simulink model "ADCS_v1"  (R2026a)
settings: Solver=VariableStepAuto  StopTime=t0  FixedStep=0.1  MaxStep=0.1
model workspace (MAT data in the model file):
  i = 8
  omega_thr = 1
  simIn : Simulink.SimulationInput (value not decoded)
  t = [0 0.1 0.2 0.3 0.4 0.5 0.6 0.7 0.8 0.9 1 1.1 ... (101 elements, 101x1)]
  u : object (value not decoded)
  y_out = [0 0 0 0 0 0 0 0]
values from neighbouring files (symbols this model uses):
  B = [1 0 0]    [parameters.m]
  h_max = 1.47    [parameters.m]
  I_RW = 1    [parameters.m]
  k_desat = 1    [parameters.m]
  kd_detumble = 1    [parameters.m]
  kd_hold = 1    [parameters.m]
  kd_point = 20    [parameters.m]
  kd_slew_fast = 1    [parameters.m]
  kd_slew_slow = 1    [parameters.m]
  kd_spin = 0    [parameters.m]
  kp_hold = 1    [parameters.m]
  kp_point = 2    [parameters.m]
  kp_slew_fast = 1    [parameters.m]
  kp_slew_slow = 1    [parameters.m]
  kp_spin = 1    [parameters.m]
  omega_0 = [0 0 0.0011]    [parameters.m]
  omega_ref = [0 0 0]    [parameters.m]
  omega_zero = 0.001    [parameters.m]
  P = satellite_params()    [individual_test_with_dynamics.m]    (also in parameters.m; test.m = thrusters(:, 1:3))
  q0 = [sqrt(0.5) -sqrt(0.5) 0 0]    [parameters.m]
  q_ref = [ cos(theta_ref/2) ... (first row only)    [parameters.m]
libraries: matrix_library x13, simulink x6, aerolibutil x4, sim3dlib x2
(part 2 of 2)

== system ADCS_v1/Subsystem2/Controller/Subsystem ==
  q_ref : Inport
  q : Inport  Port=2
  omega_ref : Inport  Port=3
  omega : Inport  Port=4
  Quaternion Inverse : aerolibutil/Quaternion Inverse
  Quaternion Multiplication : aerolibutil/Quaternion Multiplication
  Sum : Sum  Inputs=|+-
  Terminator : Terminator
  split q_error : Demux  Outputs=[1 3]
  q_err : Outport
  omega_err : Outport  Port=2
  wires:
  omega_ref/1 -> Sum/2
  omega/1 -> Sum/1
  Quaternion Inverse/1 -> Quaternion Multiplication/1
  q_ref/1 -> Quaternion Multiplication/2
  split q_error/1 -> Terminator/1
  split q_error/2 -> q_err/1
  Quaternion Multiplication/1 -> split q_error/1
  Sum/1 -> omega_err/1
  q/1 -> Quaternion Inverse/1

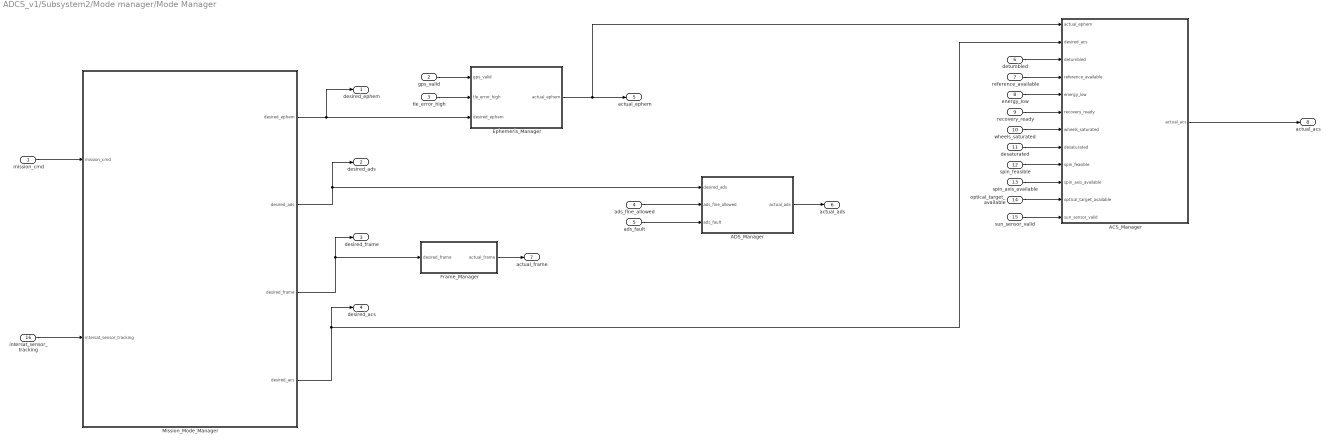
== system ADCS_v1/Subsystem2/Mode manager/Mode Manager ==
  mission_cmd : Inport  OutDataTypeStr=uint8  PortDimensions=1
  gps_valid : Inport  Port=2  OutDataTypeStr=boolean  PortDimensions=1
  tle_error_high : Inport  Port=3  OutDataTypeStr=boolean  PortDimensions=1
  ads_fine_allowed : Inport  Port=4  OutDataTypeStr=boolean  PortDimensions=1
  ads_fault : Inport  Port=5  OutDataTypeStr=boolean  PortDimensions=1
  detumbled : Inport  Port=6  OutDataTypeStr=boolean  PortDimensions=1
  reference_available : Inport  Port=7  OutDataTypeStr=boolean  PortDimensions=1
  energy_low : Inport  Port=8  OutDataTypeStr=boolean  PortDimensions=1
  recovery_ready : Inport  Port=9  OutDataTypeStr=boolean  PortDimensions=1
  wheels_saturated : Inport  Port=10  OutDataTypeStr=boolean  PortDimensions=1
  desaturated : Inport  Port=11  OutDataTypeStr=boolean  PortDimensions=1
  spin_feasible : Inport  Port=12  OutDataTypeStr=boolean  PortDimensions=1
  spin_axis_available : Inport  Port=13  OutDataTypeStr=boolean  PortDimensions=1
  optical_target_available : Inport  Port=14  OutDataTypeStr=boolean  PortDimensions=1
  sun_sensor_valid : Inport  Port=15  OutDataTypeStr=boolean  PortDimensions=1
  intersat_sensor_tracking : Inport  Port=16  OutDataTypeStr=boolean  PortDimensions=1
  ACS_Manager : Stateflow chart  TreatAsAtomicUnit=on
      settings: PortSchema="{\"entries\":[{\"content\":{\"sides\":[{\"content\":{\"connectorIds\":[\"In2\",\"In1\",\"In3\",\"In4\",\"In5\",\"In6\",\"In7\",\"In8\",\"In9\",\"In10\",\"In11\",\"In12\"]},\"type\":\"ConnectorPlacement.EquallySpacedRectSide\",\"uuid\":\"c64f5ed7-7a07-4761-a251-d625087249f8\"},{\"content\":{\"connectorIds\":[\"Out1\"],\"side\":\"RIGHT\"},\"type\":\"ConnectorPlacement.EquallySpacedRectSide\",\"uuid\":\"ff17dfa7-5a32-4799-bec0-131df3b46d45\"},{\"content\":{\"side\":\"TOP\"},\"type\":\"ConnectorPlacement.EquallySpacedRectSide\",\"uuid\":\"acaf274e-12ec-4fab-ab7e-ad580afcef6e\"}]},\"type\":\"ConnectorPlacement.EquallySpacedConnector\",\"uuid\":\"7d19de63-b993-417e-b6e9-9dc888da130b\"}],\"packageUris\":[\"http://schema.mathworks.com/mf0/Connector/R2020b\"],\"version\":\"1.0\"}"
  ADS_Manager : Stateflow chart  TreatAsAtomicUnit=on
  Ephemeris_Manager : Stateflow chart  TreatAsAtomicUnit=on
      settings: PortSchema="{\"entries\":[{\"content\":{\"sides\":[{\"content\":{\"connectorIds\":[\"In2\",\"In3\",\"In1\"]},\"type\":\"ConnectorPlacement.EquallySpacedRectSide\",\"uuid\":\"cbbccf67-8c60-498d-a98a-76db8747fb3a\"},{\"content\":{\"connectorIds\":[\"Out1\"],\"side\":\"RIGHT\"},\"type\":\"ConnectorPlacement.EquallySpacedRectSide\",\"uuid\":\"743b35d2-d398-4833-9c20-93b5e77612f2\"},{\"content\":{\"side\":\"TOP\"},\"type\":\"ConnectorPlacement.EquallySpacedRectSide\",\"uuid\":\"56075cc1-c683-438a-85bf-78d94186ffa6\"}]},\"type\":\"ConnectorPlacement.EquallySpacedConnector\",\"uuid\":\"bae867d4-09fc-4097-a23b-eff5fb3633ac\"}],\"packageUris\":[\"http://schema.mathworks.com/mf0/Connector/R2020b\"],\"version\":\"1.0\"}"
  Frame_Manager : Stateflow chart  TreatAsAtomicUnit=on
  Mission_Mode_Manager : Stateflow chart  TreatAsAtomicUnit=on
  desired_ephem : Outport
  desired_ads : Outport  Port=2
  desired_frame : Outport  Port=3
  desired_acs : Outport  Port=4
  actual_ephem : Outport  Port=5
  actual_ads : Outport  Port=6
  actual_frame : Outport  Port=7
  actual_acs : Outport  Port=8
  wires:
  spin_feasible/1 -> ACS_Manager/9(spin_feasible)
  desaturated/1 -> ACS_Manager/8(desaturated)
  spin_axis_available/1 -> ACS_Manager/10(spin_axis_available)
  mission_cmd/1 -> Mission_Mode_Manager/1(mission_cmd)
  recovery_ready/1 -> ACS_Manager/6(recovery_ready)
  ads_fault/1 -> ADS_Manager/3(ads_fault)
  intersat_sensor_tracking/1 -> Mission_Mode_Manager/2(intersat_sensor_tracking)
  gps_valid/1 -> Ephemeris_Manager/2(gps_valid)
  Ephemeris_Manager/1(actual_ephem) -> ACS_Manager/2(actual_ephem), actual_ephem/1
  ads_fine_allowed/1 -> ADS_Manager/2(ads_fine_allowed)
  ADS_Manager/1(actual_ads) -> actual_ads/1
  Mission_Mode_Manager/3(desired_frame) -> Frame_Manager/1(desired_frame), desired_frame/1
  wheels_saturated/1 -> ACS_Manager/7(wheels_saturated)
  detumbled/1 -> ACS_Manager/3(detumbled)
  reference_available/1 -> ACS_Manager/4(reference_available)
  tle_error_high/1 -> Ephemeris_Manager/3(tle_error_high)
  Mission_Mode_Manager/2(desired_ads) -> ADS_Manager/1(desired_ads), desired_ads/1
  optical_target_available/1 -> ACS_Manager/11(optical_target_available)
  Frame_Manager/1(actual_frame) -> actual_frame/1
  Mission_Mode_Manager/1(desired_ephem) -> desired_ephem/1, Ephemeris_Manager/1(desired_ephem)
  energy_low/1 -> ACS_Manager/5(energy_low)
  Mission_Mode_Manager/4(desired_acs) -> desired_acs/1, ACS_Manager/1(desired_acs)
  ACS_Manager/1(actual_acs) -> actual_acs/1
  sun_sensor_valid/1 -> ACS_Manager/12(sun_sensor_valid)

== system ADCS_v1/Subsystem1/Controller/Control Algorithms/DESAT ==
  B : Inport
  RW_omega : Inport  Port=2
  desat : ActionPort
  Cross Product : matrix_library/Cross Product
  Divide : Product  Inputs=*/
  Dot Product : DotProduct  OutDataTypeStr=Inherit: Inherit via internal rule
  Gain : Gain  Gain=-k_desat
  tau_cmd : Outport
  wires:
  B/1 -> Dot Product/1, Dot Product/2, Cross Product/2
  Divide/1 -> Gain/1
  Gain/1 -> tau_cmd/1
  Cross Product/1 -> Divide/1
  RW_omega/1 -> Cross Product/1
  Dot Product/1 -> Divide/2

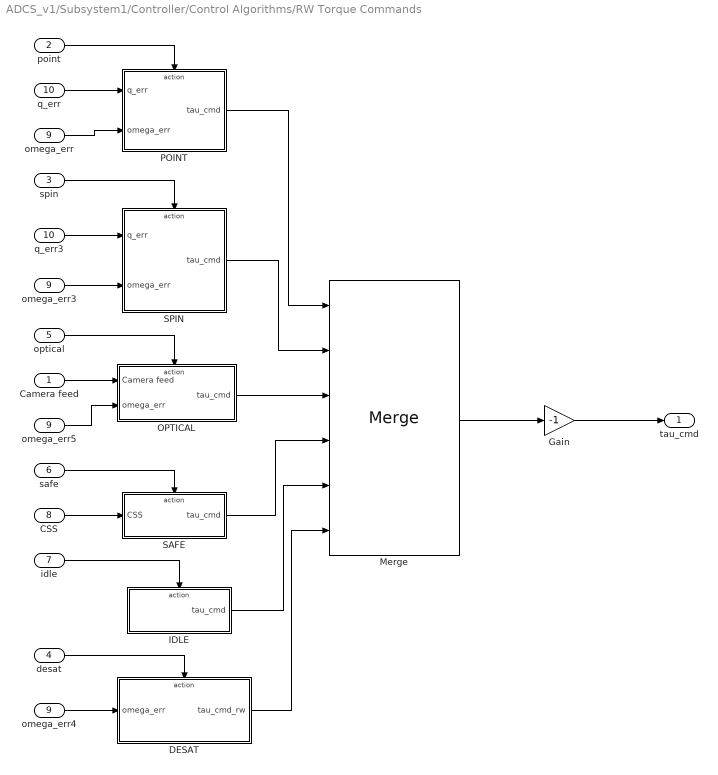
== system ADCS_v1/Subsystem1/Controller/Control Algorithms/RW Torque Commands ==
  Camera feed : Inport
  point : Inport  Port=2
  spin : Inport  Port=3
  desat : Inport  Port=4
  optical : Inport  Port=5
  safe : Inport  Port=6
  idle : Inport  Port=7
  CSS : Inport  Port=8
  omega_err : Inport  Port=9
  q_err : Inport  Port=10
  DESAT : Subsystem  TreatAsAtomicUnit=on
  Gain : Gain  Gain=-1
  IDLE : Subsystem  TreatAsAtomicUnit=on
  Merge : Merge  Inputs=6
  OPTICAL : Subsystem  TreatAsAtomicUnit=on
  POINT : Subsystem  TreatAsAtomicUnit=on
  SAFE : Subsystem  TreatAsAtomicUnit=on
  SPIN : Subsystem  TreatAsAtomicUnit=on
  omega_err3 : InportShadow  Port=9
  omega_err4 : InportShadow  Port=9
  omega_err5 : InportShadow  Port=9
  q_err3 : InportShadow  Port=10
  tau_cmd : Outport
  wires:
  idle/1 -> IDLE/Action
  spin/1 -> SPIN/Action
  Camera feed/1 -> OPTICAL/1(Camera feed)
  omega_err4/1 -> DESAT/1(omega_err)
  omega_err/1 -> POINT/2(omega_err)
  optical/1 -> OPTICAL/Action
  desat/1 -> DESAT/Action
  CSS/1 -> SAFE/1(CSS)
  point/1 -> POINT/Action
  omega_err3/1 -> SPIN/2(omega_err)
  safe/1 -> SAFE/Action
  q_err/1 -> POINT/1(q_err)
  q_err3/1 -> SPIN/1(q_err)
  omega_err5/1 -> OPTICAL/2(omega_err)
  POINT/1(tau_cmd) -> Merge/1
  SPIN/1(tau_cmd) -> Merge/2
  OPTICAL/1(tau_cmd) -> Merge/3
  SAFE/1(tau_cmd) -> Merge/4
  IDLE/1(tau_cmd) -> Merge/5
  DESAT/1(tau_cmd_rw) -> Merge/6
  Merge/1 -> Gain/1
  Gain/1 -> tau_cmd/1

== system ADCS_v1/Subsystem1/Controller/Control Algorithms/Thruster Torque commands ==
  detumble : Inport
  desat : Inport  Port=2
  default : Inport  Port=3
  omega : Inport  Port=4
  RW_omega : Inport  Port=5
  DEFAULT : Subsystem  TreatAsAtomicUnit=on
  DESAT : Subsystem  TreatAsAtomicUnit=on
  DETUMBLE : Subsystem  TreatAsAtomicUnit=on
  Merge1 : Merge  Inputs=3
  tau_cmd : Outport
  wires:
  omega/1 -> DETUMBLE/1(omega)
  DETUMBLE/1(tau_cmd) -> Merge1/1
  Merge1/1 -> tau_cmd/1
  detumble/1 -> DETUMBLE/Action
  default/1 -> DEFAULT/Action
  DEFAULT/1(tau_cmd) -> Merge1/3
  RW_omega/1 -> DESAT/1(RW_omega)
  desat/1 -> DESAT/Action
  DESAT/1(tau_cmd) -> Merge1/2

== system ADCS_v1/Subsystem1/Controller/Control Algorithms/default ==
  detumble : ActionPort
  Constant : Constant  Value=[0 0 0]
  tau_cmd : Outport
  wires:
  Constant/1 -> tau_cmd/1

== system ADCS_v1/Subsystem1/Subsystem/LVLH/norm ==
  In1 : Inport
  Sqrt : Sqrt
  Square : Math  Operator=square
  Sum of Elements : Sum  Inputs=+
  Out1 : Outport
  wires:
  In1/1 -> Square/1
  Square/1 -> Sum of Elements/1
  Sum of Elements/1 -> Sqrt/1
  Sqrt/1 -> Out1/1

== system ADCS_v1/Subsystem1/Subsystem/LVLH/norm1 ==
  In1 : Inport
  Sqrt : Sqrt
  Square : Math  Operator=square
  Sum of Elements : Sum  Inputs=+
  Out1 : Outport
  wires:
  Sqrt/1 -> Out1/1
  Sum of Elements/1 -> Sqrt/1
  Square/1 -> Sum of Elements/1
  In1/1 -> Square/1

== system ADCS_v1/Subsystem1/Subsystem/Sun_point/Pointing_r ==
  v_si : Inport
  r_si : Inport  Port=2
  v_sun_i : Inport  Port=3
  r_sun_i : Inport  Port=4
  Sum : Sum  Inputs=|-+
  Sum1 : Sum  Inputs=|-+
  v_point : Outport
  r_point : Outport  Port=2
  wires:
  Sum1/1 -> v_point/1
  v_si/1 -> Sum1/1
  Sum/1 -> r_point/1
  r_si/1 -> Sum/1
  v_sun_i/1 -> Sum1/2
  r_sun_i/1 -> Sum/2

== system ADCS_v1/Subsystem1/Subsystem/Sun_point/norm ==
  r_point : Inport
  Sqrt : Sqrt
  Square : Math  Operator=square
  Sum of Elements : Sum  Inputs=+
  Out1 : Outport
  wires:
  r_point/1 -> Square/1
  Square/1 -> Sum of Elements/1
  Sum of Elements/1 -> Sqrt/1
  Sqrt/1 -> Out1/1

== system ADCS_v1/Subsystem1/Subsystem/Sun_point/norm1 ==
  In1 : Inport
  Sqrt : Sqrt
  Square : Math  Operator=square
  Sum of Elements : Sum  Inputs=+
  Out1 : Outport
  wires:
  Sqrt/1 -> Out1/1
  Sum of Elements/1 -> Sqrt/1
  Square/1 -> Sum of Elements/1
  In1/1 -> Square/1

== system ADCS_v1/Subsystem1/Subsystem/Target_Pointing/Pointing_r ==
  v_si : Inport
  r_si : Inport  Port=2
  r_pi : Inport  Port=3
  Sum : Sum  Inputs=-+|
  Sum1 : Sum  Inputs=|-+
  omega_E : Constant  Value=[0 0 7.2921159e-5]
  v_p : matrix_library/Cross Product
  v_point : Outport
  r_point : Outport  Port=2
  wires:
  r_si/1 -> Sum/1
  r_pi/1 -> v_p/2, Sum/2
  Sum/1 -> r_point/1
  v_si/1 -> Sum1/1
  omega_E/1 -> v_p/1
  Sum1/1 -> v_point/1
  v_p/1 -> Sum1/2

== system ADCS_v1/Subsystem1/Subsystem/Target_Pointing/norm ==
  r_point : Inport
  Sqrt : Sqrt
  Square : Math  Operator=square
  Sum of Elements : Sum  Inputs=+
  Out1 : Outport
  wires:
  Sqrt/1 -> Out1/1
  Sum of Elements/1 -> Sqrt/1
  Square/1 -> Sum of Elements/1
  r_point/1 -> Square/1

== system ADCS_v1/Subsystem1/Subsystem/Target_Pointing/norm1 ==
  In1 : Inport
  Sqrt : Sqrt
  Square : Math  Operator=square
  Sum of Elements : Sum  Inputs=+
  Out1 : Outport
  wires:
  In1/1 -> Square/1
  Square/1 -> Sum of Elements/1
  Sum of Elements/1 -> Sqrt/1
  Sqrt/1 -> Out1/1

== system ADCS_v1/Subsystem1/Subsystem/VNB/Subsystem ==
  In1 : Inport
  Default : Subsystem  TreatAsAtomicUnit=on
  M_MAX_DRAG : Subsystem  TreatAsAtomicUnit=on
  M_MIN_DRAG : Subsystem  TreatAsAtomicUnit=on
  M_RAM : Subsystem  TreatAsAtomicUnit=on
  Merge : Merge  Inputs=4
  Switch Case : SwitchCase  CaseConditions={8,9,10}
  Out3 : Outport
  wires:
  Switch Case/1 -> M_MIN_DRAG/Action
  In1/1 -> Switch Case/1
  Switch Case/4 -> Default/Action
  Switch Case/3 -> M_RAM/Action
  Switch Case/2 -> M_MAX_DRAG/Action
  Merge/1 -> Out3/1
  M_MIN_DRAG/1(Out1) -> Merge/1
  M_MAX_DRAG/1(Out1) -> Merge/2
  M_RAM/1(Out1) -> Merge/3
  Default/1(Out1) -> Merge/4

== system ADCS_v1/Subsystem1/Subsystem/VNB/norm ==
  In1 : Inport
  Sqrt : Sqrt
  Square : Math  Operator=square
  Sum of Elements : Sum  Inputs=+
  Out1 : Outport
  wires:
  In1/1 -> Square/1
  Square/1 -> Sum of Elements/1
  Sum of Elements/1 -> Sqrt/1
  Sqrt/1 -> Out1/1

== system ADCS_v1/Subsystem1/Subsystem/VNB/norm2 ==
  v_s : Inport
  Sqrt : Sqrt
  Square : Math  Operator=square
  Sum of Elements : Sum  Inputs=+
  Out1 : Outport
  wires:
  Sqrt/1 -> Out1/1
  Sum of Elements/1 -> Sqrt/1
  Square/1 -> Sum of Elements/1
  v_s/1 -> Square/1

== system ADCS_v1/Subsystem1/Subsystem/VNB/norm3 ==
  , : Inport
  Sqrt : Sqrt
  Square : Math  Operator=square
  Sum of Elements : Sum  Inputs=+
  Out1 : Outport
  wires:
  Sqrt/1 -> Out1/1
  Sum of Elements/1 -> Sqrt/1
  Square/1 -> Sum of Elements/1
  ,/1 -> Square/1

== system ADCS_v1/Subsystem2/Controller/Control Algorithms/DESAT ==
  B : Inport
  RW_omega : Inport  Port=2
  desat : ActionPort
  Cross Product : matrix_library/Cross Product
  Divide : Product  Inputs=*/
  Dot Product : DotProduct  OutDataTypeStr=Inherit: Inherit via internal rule
  Gain : Gain  Gain=k_desat
  tau_cmd : Outport
  wires:
  Dot Product/1 -> Divide/2
  RW_omega/1 -> Cross Product/1
  Cross Product/1 -> Divide/1
  Gain/1 -> tau_cmd/1
  Divide/1 -> Gain/1
  B/1 -> Cross Product/2, Dot Product/2, Dot Product/1

== system ADCS_v1/Subsystem2/Controller/Control Algorithms/DETUMBLE1 ==
  detumble : ActionPort
  Constant : Constant  Value=[0 0 0]
  tau_cmd : Outport
  wires:
  Constant/1 -> tau_cmd/1

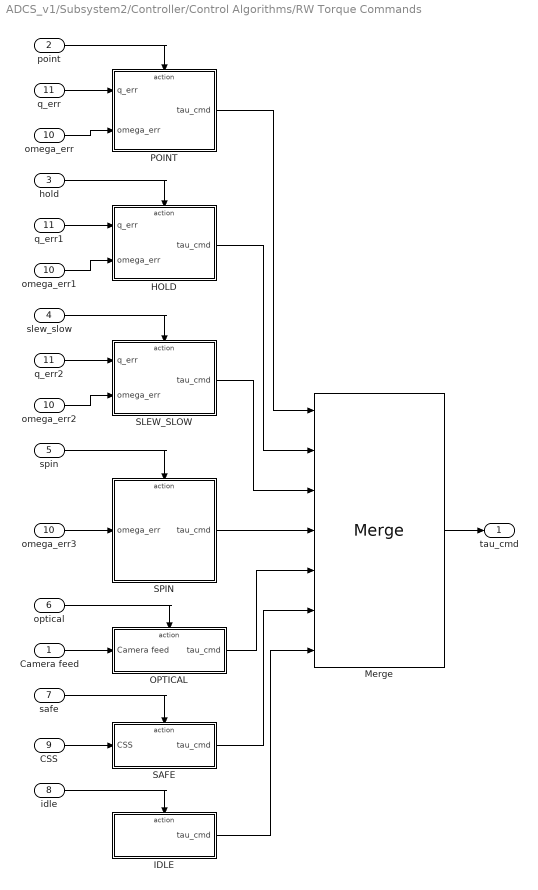
== system ADCS_v1/Subsystem2/Controller/Control Algorithms/RW Torque Commands ==
  Camera feed : Inport
  point : Inport  Port=2
  hold : Inport  Port=3
  slew_slow : Inport  Port=4
  spin : Inport  Port=5
  optical : Inport  Port=6
  safe : Inport  Port=7
  idle : Inport  Port=8
  CSS : Inport  Port=9
  omega_err : Inport  Port=10
  q_err : Inport  Port=11
  HOLD : Subsystem  TreatAsAtomicUnit=on
  IDLE : Subsystem  TreatAsAtomicUnit=on
  Merge : Merge  Inputs=7
  OPTICAL : Subsystem  TreatAsAtomicUnit=on
  POINT : Subsystem  TreatAsAtomicUnit=on
  SAFE : Subsystem  TreatAsAtomicUnit=on
  SLEW_SLOW : Subsystem  TreatAsAtomicUnit=on
  SPIN : Subsystem  TreatAsAtomicUnit=on
  omega_err1 : InportShadow  Port=10
  omega_err2 : InportShadow  Port=10
  omega_err3 : InportShadow  Port=10
  q_err1 : InportShadow  Port=11
  q_err2 : InportShadow  Port=11
  tau_cmd : Outport
  wires:
  Merge/1 -> tau_cmd/1
  IDLE/1(tau_cmd) -> Merge/7
  SAFE/1(tau_cmd) -> Merge/6
  OPTICAL/1(tau_cmd) -> Merge/5
  SPIN/1(tau_cmd) -> Merge/4
  HOLD/1(tau_cmd) -> Merge/2
  POINT/1(tau_cmd) -> Merge/1
  idle/1 -> IDLE/Action
  CSS/1 -> SAFE/1(CSS)
  Camera feed/1 -> OPTICAL/1(Camera feed)
  optical/1 -> OPTICAL/Action
  omega_err3/1 -> SPIN/1(omega_err)
  spin/1 -> SPIN/Action
  omega_err2/1 -> SLEW_SLOW/2(omega_err)
  q_err2/1 -> SLEW_SLOW/1(q_err)
  omega_err1/1 -> HOLD/2(omega_err)
  q_err/1 -> POINT/1(q_err)
  omega_err/1 -> POINT/2(omega_err)
  q_err1/1 -> HOLD/1(q_err)
  point/1 -> POINT/Action
  SLEW_SLOW/1(tau_cmd) -> Merge/3
  hold/1 -> HOLD/Action
  slew_slow/1 -> SLEW_SLOW/Action
  safe/1 -> SAFE/Action

== system ADCS_v1/Subsystem2/Controller/Control Algorithms/Thruster Torque commands ==
  detumble : Inport
  slew_fast : Inport  Port=2
  default : Inport  Port=3
  omega : Inport  Port=4
  q_err : Inport  Port=5
  omega_err : Inport  Port=6
  DEFAULT : Subsystem  TreatAsAtomicUnit=on
  DETUMBLE : Subsystem  TreatAsAtomicUnit=on
  Merge1 : Merge  Inputs=3
  SLEW_FAST : Subsystem  TreatAsAtomicUnit=on
  tau_cmd : Outport
  wires:
  default/1 -> DEFAULT/Action
  detumble/1 -> DETUMBLE/Action
  slew_fast/1 -> SLEW_FAST/Action
  omega_err/1 -> SLEW_FAST/2(omega_err)
  q_err/1 -> SLEW_FAST/1(q_err)
  Merge1/1 -> tau_cmd/1
  DEFAULT/1(tau_cmd) -> Merge1/3
  DETUMBLE/1(tau_cmd) -> Merge1/1
  omega/1 -> DETUMBLE/1(omega)
  SLEW_FAST/1(tau_cmd) -> Merge1/2

== system ADCS_v1/Subsystem1/Controller/Control Algorithms/RW Torque Commands/DESAT ==
  omega_err : Inport
  desat : ActionPort
  Gain1 : Gain  Gain=-kd_point
  tau_cmd_rw : Outport
  wires:
  omega_err/1 -> Gain1/1
  Gain1/1 -> tau_cmd_rw/1

== system ADCS_v1/Subsystem1/Controller/Control Algorithms/RW Torque Commands/IDLE ==
  idle : ActionPort
  Constant : Constant  Value=[0 0 0]
  tau_cmd : Outport
  wires:
  Constant/1 -> tau_cmd/1

== system ADCS_v1/Subsystem1/Controller/Control Algorithms/RW Torque Commands/OPTICAL ==
  Camera feed : Inport
  omega_err : Inport  Port=2
  optical : ActionPort
  Constant1 : Constant  Value=0
  Gain1 : Gain  Gain=kd_point
  Gain2 : Gain  Gain=kp_point*0.005
  Gain3 : Gain  Gain=-1
  MATLAB Function2 : MATLAB Function  TreatAsAtomicUnit=on
  Mux : Mux  Inputs=3
  Sum1 : Sum  Inputs=|+-
  tau_cmd : Outport
  wires:
  Camera feed/1 -> MATLAB Function2/1(u)
  Gain1/1 -> Sum1/2
  Sum1/1 -> tau_cmd/1
  Mux/1 -> Gain2/1
  Gain2/1 -> Sum1/1
  Constant1/1 -> Mux/3
  MATLAB Function2/2(x_cm) -> Mux/2
  omega_err/1 -> Gain1/1
  MATLAB Function2/1(y_cm) -> Gain3/1
  Gain3/1 -> Mux/1

== system ADCS_v1/Subsystem1/Controller/Control Algorithms/RW Torque Commands/POINT ==
  q_err : Inport
  omega_err : Inport  Port=2
  point : ActionPort
  Gain : Gain  Gain=-kd_point
  Gain1 : Gain  Gain=kp_point
  Sum : Sum  Inputs=|++
  tau_cmd : Outport
  wires:
  Sum/1 -> tau_cmd/1
  omega_err/1 -> Gain/1
  Gain1/1 -> Sum/1
  Gain/1 -> Sum/2
  q_err/1 -> Gain1/1

== system ADCS_v1/Subsystem1/Controller/Control Algorithms/RW Torque Commands/SAFE ==
  CSS : Inport
  safe : ActionPort
  Constant : Constant  Value=[0 0 0]
  tau_cmd : Outport
  wires:
  Constant/1 -> tau_cmd/1

== system ADCS_v1/Subsystem1/Controller/Control Algorithms/RW Torque Commands/SPIN ==
  q_err : Inport
  omega_err : Inport  Port=2
  spin : ActionPort
  Constant : Constant  Value=[0 0 1]
  Constant1 : Constant  Value=[1 1 1]
  Gain : Gain  Gain=kd_spin
  Gain1 : Gain  Gain=kp_spin
  Gain2 : Gain  Gain=0.04
  Product : Product
  Sum : Sum  Inputs=|+-
  Sum1 : Sum  Inputs=|+-
  Sum2 : Sum  Inputs=|+-
  tau_cmd : Outport
  wires:
  Sum/1 -> Gain/1
  omega_err/1 -> Sum/1
  Constant/1 -> Sum2/2, Gain2/1
  Gain/1 -> Sum1/2
  Sum1/1 -> tau_cmd/1
  Constant1/1 -> Sum2/1
  q_err/1 -> Product/1
  Sum2/1 -> Product/2
  Product/1 -> Gain1/1
  Gain1/1 -> Sum1/1
  Gain2/1 -> Sum/2

== system ADCS_v1/Subsystem1/Controller/Control Algorithms/Thruster Torque commands/DEFAULT ==
  default : ActionPort
  Constant : Constant  Value=[0 0 0]
  tau_cmd : Outport
  wires:
  Constant/1 -> tau_cmd/1

== system ADCS_v1/Subsystem1/Controller/Control Algorithms/Thruster Torque commands/DESAT ==
  RW_omega : Inport
  desat : ActionPort
  Gain2 : Gain  Gain=-k_desat
  tau_cmd : Outport
  wires:
  RW_omega/1 -> Gain2/1
  Gain2/1 -> tau_cmd/1

== system ADCS_v1/Subsystem1/Controller/Control Algorithms/Thruster Torque commands/DETUMBLE ==
  omega : Inport
  detumble : ActionPort
  Gain : Gain  Gain=-kd_detumble
  tau_cmd : Outport
  wires:
  omega/1 -> Gain/1
  Gain/1 -> tau_cmd/1

== system ADCS_v1/Subsystem1/Subsystem/VNB/Subsystem/Default ==
  min drag : ActionPort
  Constant : Constant  Value=[1 0 0; 0 1 0; 0 0 1]
  Out1 : Outport
  wires:
  Constant/1 -> Out1/1

== system ADCS_v1/Subsystem1/Subsystem/VNB/Subsystem/M_MAX_DRAG ==
  max drag : ActionPort
  Constant : Constant  Value=[0 0 1; 0 1 0; -1 0 0]
  Out1 : Outport
  wires:
  Constant/1 -> Out1/1

== system ADCS_v1/Subsystem1/Subsystem/VNB/Subsystem/M_MIN_DRAG ==
  min drag : ActionPort
  Constant : Constant  Value=[1 0 0; 0 1 0; 0 0 1]
  Out1 : Outport
  wires:
  Constant/1 -> Out1/1

== system ADCS_v1/Subsystem1/Subsystem/VNB/Subsystem/M_RAM ==
  RAM : ActionPort
  Constant1 : Constant  Value=[0 0 1; 0 1 0; -1 0 0]
  Out1 : Outport
  wires:
  Constant1/1 -> Out1/1

== system ADCS_v1/Subsystem2/Controller/Control Algorithms/RW Torque Commands/HOLD ==
  q_err : Inport
  omega_err : Inport  Port=2
  hold : ActionPort
  Gain : Gain  Gain=kd_hold
  Gain1 : Gain  Gain=kp_hold
  Sum : Sum  Inputs=|++
  tau_cmd : Outport
  wires:
  Gain/1 -> Sum/2
  omega_err/1 -> Gain/1
  Sum/1 -> tau_cmd/1
  Gain1/1 -> Sum/1
  q_err/1 -> Gain1/1

== system ADCS_v1/Subsystem2/Controller/Control Algorithms/RW Torque Commands/IDLE ==
  idle : ActionPort
  Constant : Constant  Value=[0 0 0]
  tau_cmd : Outport
  wires:
  Constant/1 -> tau_cmd/1

== system ADCS_v1/Subsystem2/Controller/Control Algorithms/RW Torque Commands/OPTICAL ==
  Camera feed : Inport
  optical : ActionPort
  Constant : Constant  Value=[0 0 0]
  tau_cmd : Outport
  wires:
  Constant/1 -> tau_cmd/1

== system ADCS_v1/Subsystem2/Controller/Control Algorithms/RW Torque Commands/POINT ==
  q_err : Inport
  omega_err : Inport  Port=2
  point : ActionPort
  Gain : Gain  Gain=kd_point
  Gain1 : Gain  Gain=kp_point
  Sum : Sum  Inputs=|++
  tau_cmd : Outport
  wires:
  Gain/1 -> Sum/2
  Gain1/1 -> Sum/1
  q_err/1 -> Gain1/1
  omega_err/1 -> Gain/1
  Sum/1 -> tau_cmd/1

== system ADCS_v1/Subsystem2/Controller/Control Algorithms/RW Torque Commands/SAFE ==
  CSS : Inport
  safe : ActionPort
  Constant : Constant  Value=[0 0 0]
  tau_cmd : Outport
  wires:
  Constant/1 -> tau_cmd/1

== system ADCS_v1/Subsystem2/Controller/Control Algorithms/RW Torque Commands/SLEW_SLOW ==
  q_err : Inport
  omega_err : Inport  Port=2
  slew_slow : ActionPort
  Gain : Gain  Gain=kd_slew_slow
  Gain1 : Gain  Gain=kp_slew_slow
  Sum : Sum  Inputs=|++
  tau_cmd : Outport
  wires:
  q_err/1 -> Gain1/1
  Gain1/1 -> Sum/1
  Sum/1 -> tau_cmd/1
  omega_err/1 -> Gain/1
  Gain/1 -> Sum/2

== system ADCS_v1/Subsystem2/Controller/Control Algorithms/RW Torque Commands/SPIN ==
  omega_err : Inport
  spin : ActionPort
  Gain : Gain  Gain=kd_spin
  tau_cmd : Outport
  wires:
  omega_err/1 -> Gain/1
  Gain/1 -> tau_cmd/1

== system ADCS_v1/Subsystem2/Controller/Control Algorithms/Thruster Torque commands/DEFAULT ==
  default : ActionPort
  Constant : Constant  Value=[0 0 0]
  tau_cmd : Outport
  wires:
  Constant/1 -> tau_cmd/1

== system ADCS_v1/Subsystem2/Controller/Control Algorithms/Thruster Torque commands/DETUMBLE ==
  omega : Inport
  detumble : ActionPort
  Gain : Gain  Gain=kd_detumble
  tau_cmd : Outport
  wires:
  Gain/1 -> tau_cmd/1
  omega/1 -> Gain/1

== system ADCS_v1/Subsystem2/Controller/Control Algorithms/Thruster Torque commands/SLEW_FAST ==
  q_err : Inport
  omega_err : Inport  Port=2
  slew_fast : ActionPort
  Gain : Gain  Gain=kd_slew_fast
  Gain1 : Gain  Gain=kp_slew_fast
  Sum : Sum  Inputs=|++
  tau_cmd : Outport
  wires:
  q_err/1 -> Gain1/1
  Gain1/1 -> Sum/1
  Sum/1 -> tau_cmd/1
  omega_err/1 -> Gain/1
  Gain/1 -> Sum/2

== stateflow chart ADCS_v1/Subsystem1/Mode manager/Mode Manager/ADS_Manager ==
  state ADS_IDLE
    entry:
    actual_ads = uint8(0);
  state ADS_UKF_FINE
    entry:
    actual_ads = uint8(2);
  state ADS_UKF_COARSE
    entry:
    actual_ads = uint8(1);
  ADS_UKF_FINE -> ADS_IDLE [order 2] : [desired_ads == uint8(0) || ads_fault]
  ADS_IDLE -> ADS_UKF_FINE [order 2] : [desired_ads == uint8(2) &&...
      |  ads_fine_allowed && ~ads_fault]
  (default) -> ADS_IDLE
  ADS_UKF_COARSE -> ADS_IDLE [order 1] : [desired_ads == uint8(0) || ads_fault]
  ADS_IDLE -> ADS_UKF_COARSE [order 1] : [desired_ads == uint8(1) ||...
      |  (desired_ads == uint8(2) &&...
      |  ~ads_fine_allowed)]
  ADS_UKF_FINE -> ADS_UKF_COARSE [order 1] : [desired_ads == uint8(1) ||...
      |  ~ads_fine_allowed]
  ADS_UKF_COARSE -> ADS_UKF_FINE [order 2] : [desired_ads == uint8(2) &&...
      |  ads_fine_allowed && ~ads_fault]
  data: desired_ads input uint8; ads_fine_allowed input boolean; ads_fault input boolean; actual_ads output uint8 =0

== stateflow chart ADCS_v1/Subsystem1/Mode manager/Mode Manager/Ephemeris_Manager ==
  state EPHEM_IDLE
    entry:
    actual_ephem = uint8(0);
  state EPHEM_GPS
    entry:
    actual_ephem = uint8(2);
  state EPHEM_TLE
    entry:
    actual_ephem = uint8(1);
  EPHEM_GPS -> EPHEM_IDLE [order 1] : [desired_ephem == uint8(0)]
  EPHEM_IDLE -> EPHEM_GPS [order 2] : [desired_ephem == uint8(2)...
      |  && gps_valid]
  (default) -> EPHEM_IDLE
  EPHEM_IDLE -> EPHEM_TLE [order 1] : [desired_ephem == uint8(1) ||...
      |  (desired_ephem == uint8(2) &&...
      |  ~gps_valid && ~tle_error_high)]
  EPHEM_TLE -> EPHEM_IDLE [order 1] : [desired_ephem == uint8(0)...
      |  || tle_error_high]
  EPHEM_GPS -> EPHEM_TLE [order 2] : [desired_ephem == uint8(1) ||...
      |  ~gps_valid]
  EPHEM_TLE -> EPHEM_GPS [order 2] : [desired_ephem == uint8(2) && gps_valid]
  data: desired_ephem input uint8; gps_valid input boolean; tle_error_high input boolean; actual_ephem output uint8 =0

== stateflow chart ADCS_v1/Subsystem1/Mode manager/Mode Manager/Frame_Manager ==
  state FRAME_INERTIAL
    entry:
    actual_frame = uint8(2);
  state FRAME_LVLH
    entry:
    actual_frame = uint8(3);
  state FRAME_BODY
    entry:
    actual_frame = uint8(1);
  state FRAME_EARTH_TARGET
    entry:
    actual_frame = uint8(4);
  state FRAME_IDLE
    entry:
    actual_frame = uint8(0);
  state FRAME_IMAGING_TDI
    entry:
    actual_frame = uint8(6);
  state FRAME_VNB
    entry:
    actual_frame = uint8(5);
  FRAME_INERTIAL -> (junction 11) : [desired_frame ~= uint8(2)]
  (junction 11) -> FRAME_INERTIAL [order 3] : [desired_frame == uint8(2)]
  FRAME_LVLH -> (junction 11) : [desired_frame ~= uint8(3)]
  (junction 11) -> FRAME_LVLH [order 4] : [desired_frame == uint8(3)]
  FRAME_BODY -> (junction 11) : [desired_frame ~= uint8(1)]
  (junction 11) -> FRAME_BODY [order 2] : [desired_frame == uint8(1)]
  FRAME_EARTH_TARGET -> (junction 11) : [desired_frame ~= uint8(4)]
  (junction 11) -> FRAME_EARTH_TARGET [order 5] : [desired_frame == uint8(4)]
  (junction 11) -> FRAME_IDLE [order 1] : [desired_frame == uint8(0)]
  FRAME_IDLE -> (junction 11) : [desired_frame ~= uint8(0)]
  FRAME_IMAGING_TDI -> (junction 11) : [desired_frame ~= uint8(6)]
  (junction 11) -> FRAME_VNB [order 6] : [desired_frame == uint8(5)]
  (junction 11) -> FRAME_IMAGING_TDI [order 7] : [desired_frame == uint8(6)]
  FRAME_VNB -> (junction 11) : [desired_frame ~= uint8(5)]
  (default) -> FRAME_IDLE
  data: desired_frame input uint8; actual_frame output uint8 =0

== stateflow chart ADCS_v1/Subsystem1/Mode manager/Mode Manager/Mission_Mode_Manager ==
  state M_DETUMBLE
    entry:
    desired_ephem = uint8(0);
    desired_ads = uint8(1);
    desired_frame = uint8(0);
    desired_acs = uint8(1);
    %desired_actuator = uint8(3);
  state M_SAFE_SUN
    entry:
    desired_ephem = uint8(0);
    desired_ads = uint8(0);
    desired_frame = uint8(0);
    desired_acs = uint8(6);
    %desired_actuator = uint8(2);
  state M_Y_SPIN
    entry:
    desired_ephem = uint8(2);
    desired_ads = uint8(1);
    desired_frame = uint8(1);
    desired_acs = uint8(3);
    %desired_actuator = uint8(2);
  state M_IDLE
    entry:
    desired_ephem = uint8(0);
    desired_ads = uint8(0);
    desired_frame = uint8(0);
    desired_acs = uint8(0);
    %desired_actuator = uint8(0);
  state M_MIN_DRAG
    entry:
    desired_ephem = uint8(2);
    desired_ads = uint8(2);
    desired_frame = uint8(5);
    desired_acs = uint8(2);
    %desired_actuator = uint8(2);
  state M_POINT_NADIR
    entry:
    desired_ephem = uint8(2);
    desired_ads = uint8(2);
    desired_frame = uint8(3);
    desired_acs = uint8(2);
    %desired_actuator = uint8(2);
  state M_MAX_DRAG
    entry:
    desired_ephem = uint8(2);
    desired_ads = uint8(2);
    desired_frame = uint8(5);
    desired_acs = uint8(2);
    %desired_actuator = uint8(2);
  state M_POINT_EARTH_TARGET
    entry:
    desired_ephem = uint8(2);
    desired_ads = uint8(2);
    desired_frame = uint8(4);
    desired_acs = uint8(2);
    %desired_actuator = uint8(2);
  state M_RAM
    entry:
    desired_ephem = uint8(2);
    desired_ads = uint8(2);
    desired_frame = uint8(5);
    desired_acs = uint8(2);
    %desired_actuator = uint8(2);
  state M_POINT_SUN
    entry:
    desired_ephem = uint8(2);
    desired_ads = uint8(2);
    desired_frame = uint8(2);
    desired_acs = uint8(2);
    %desired_actuator = uint8(2);
  state M_INTERSAT_TRACK
    entry:
    desired_ephem = uint8(2);
    desired_ads = uint8(2);
    desired_frame = uint8(2);
    desired_acs = uint8(5);
    %desired_actuator = uint8(2);
  M_DETUMBLE -> (junction 28) : [mission_cmd ~= uint8(1)]
  (junction 28) -> M_DETUMBLE [order 3] : [mission_cmd == uint8(1)]
  M_Y_SPIN -> (junction 28) : [mission_cmd ~= uint8(3)]
  M_SAFE_SUN -> (junction 28) : [mission_cmd ~= uint8(2)]
  (junction 28) -> M_SAFE_SUN [order 4] : [mission_cmd == uint8(2)]
  M_IDLE -> (junction 28) : [mission_cmd ~= uint8(0)]
  (default) -> M_IDLE
  (junction 28) -> M_IDLE [order 1] : [mission_cmd == uint8(0)]
  (junction 28) -> M_Y_SPIN [order 5] : [mission_cmd == uint8(3)]
  (junction 28) -> M_MIN_DRAG [order 11] : [mission_cmd == uint8(8)]
  M_MIN_DRAG -> (junction 28) : [mission_cmd ~= uint8(8)]
  (junction 28) -> M_POINT_NADIR [order 6] : [mission_cmd == uint8(4)]
  M_POINT_NADIR -> (junction 28) : [mission_cmd ~= uint8(4)]
  (junction 28) -> M_MAX_DRAG [order 2] : [mission_cmd == uint8(9)]
  M_MAX_DRAG -> (junction 28) : [mission_cmd ~= uint8(9)]
  (junction 28) -> M_POINT_EARTH_TARGET [order 8] : [mission_cmd == uint8(6)]
  (junction 28) -> M_POINT_SUN [order 7] : [mission_cmd == uint8(5)]
  M_POINT_EARTH_TARGET -> (junction 28) : [mission_cmd ~= uint8(6)]
  M_POINT_SUN -> (junction 28) : [mission_cmd ~= uint8(5)]
  (junction 28) -> M_INTERSAT_TRACK [order 9] : [mission_cmd == uint8(7)]
  (junction 28) -> M_RAM [order 10] : [mission_cmd == uint8(10)]
  M_INTERSAT_TRACK -> (junction 28) : [mission_cmd ~= uint8(7)]
  M_RAM -> (junction 28) : [mission_cmd ~= uint8(10)]
  data: mission_cmd input uint8; intersat_sensor_tracking input boolean; desired_ephem output uint8 =0; desired_ads output uint8 =0; desired_frame output uint8 =0; desired_acs output uint8 =0

== stateflow chart ADCS_v1/Subsystem1/Mode manager/Status_Manager ==
  state STATUS
    during:
    mode_degraded = (actual_ephem ~= desired_ephem) || (actual_ads ~= desired_ads) || (actual_frame ~= desired_frame) || (actual_acs ~= desired_acs);
  (default) -> STATUS
  data: desired_ephem input uint8; desired_ads input uint8; desired_frame input uint8; desired_acs input uint8; actual_ephem input uint8; actual_ads input uint8; actual_frame input uint8; actual_acs input uint8; mode_degraded output boolean =0

== stateflow chart ADCS_v1/Subsystem2/Mode manager/Mode Manager/ACS_Manager ==
  state ACS_DETUMBLE
    entry:
    actual_acs = uint8(1);
  state ACS_POINT
    entry:
    actual_acs = uint8(2);
  state ACS_IDLE
    entry:
    actual_acs = uint8(0);
  state ACS_SLEW_SLOW
    entry:
    actual_acs = uint8(4);
  state ACS_DESAT
    entry:
    actual_acs = uint8(7);
    %exit:
    %desaturated = 1;
  state ACS_HOLD
    entry:
    actual_acs = uint8(3);
  state ACS_OPTICAL
    entry:
    actual_acs = uint8(8);
  state ACS_SPIN
    entry:
    actual_acs = uint8(6);
  state ACS_SLEW_FAST
    entry:
    actual_acs = uint8(5);
  state ACS_SAFE
    entry:
    actual_acs = uint8(9);
  ACS_SLEW_SLOW -> ACS_DESAT [order 3] : [wheels_saturated && ~energy_low]
  ACS_OPTICAL -> ACS_POINT [order 3] : [~optical_target_available &&...
      |  ~energy_low]
  (junction 25) -> ACS_DETUMBLE [order 2] : [desired_acs == uint8(1)]
  ACS_DETUMBLE -> (junction 25) : [desired_acs ~= uint8(1)]
  ACS_POINT -> ACS_SAFE [order 2] : [energy_low || ~reference_available ||...
      |  ~detumbled || actual_ephem == uint8(0)]
  (junction 25) -> ACS_IDLE [order 1] : [desired_acs == uint8(0)]
  ACS_POINT -> (junction 25) [order 1] : [desired_acs ~= uint8(2) &&...
      |  ~(desired_acs == uint8(8) &&...
      |  ~optical_target_available)]
  (junction 25) -> ACS_POINT [order 3] : [desired_acs == uint8(2)]
  (default) -> ACS_IDLE
  ACS_IDLE -> (junction 25) : [desired_acs ~= uint8(0)]
  (junction 25) -> ACS_SLEW_SLOW [order 5] : [desired_acs == uint8(4)]
  ACS_SLEW_SLOW -> (junction 25) [order 1] : [desired_acs ~= uint8(4)]
  ACS_SLEW_SLOW -> ACS_SAFE [order 2] : [energy_low || ~detumbled ||...
      |  actual_ephem == uint8(0)]
  ACS_HOLD -> (junction 25) [order 1] : [desired_acs ~= uint8(3)]
  ACS_DESAT -> (junction 25) [order 1] : [desired_acs ~= uint8(7) &&...
      |  desaturated && recovery_ready &&...
      |  ~energy_low]
  (junction 25) -> ACS_HOLD [order 4] : [desired_acs == uint8(3)]
  (junction 25) -> ACS_DESAT [order 8] : [desired_acs == uint8(7)]
  ACS_OPTICAL -> (junction 25) [order 1] : [desired_acs ~= uint8(8) && optical_target_available]
  (junction 25) -> ACS_OPTICAL [order 9] : [desired_acs == uint8(8)]
  (junction 25) -> ACS_SLEW_FAST [order 6] : [desired_acs == uint8(5)]
  ACS_SLEW_FAST -> (junction 25) [order 1] : [desired_acs ~= uint8(5)]
  ACS_SAFE -> (junction 25) : [desired_acs ~= uint8(9) &&...
      |  ~energy_low && recovery_ready &&...
      |  sun_sensor_valid && ~((desired_acs == uint8(2)) &&...
      |  ~reference_available) && ~((desired_acs == uint8(6)) &&...
      |  (~spin_feasible || ~spin_axis_available))]
  (junction 25) -> ACS_SAFE [order 10] : [desired_acs == uint8(9)]
  (junction 25) -> ACS_SPIN [order 7] : [desired_acs == uint8(6)]
  ACS_SPIN -> (junction 25) [order 2] : [desired_acs ~= uint8(6)]
  ACS_DESAT -> ACS_SAFE [order 2] : [energy_low]
  ACS_SLEW_FAST -> ACS_DESAT [order 3] : [wheels_saturated && ~energy_low]
  ACS_HOLD -> ACS_SAFE [order 2] : [energy_low ||...
      |  ~detumbled ||...
      |  actual_ephem == uint8(0)]
  ACS_OPTICAL -> ACS_SAFE [order 2] : [energy_low]
  ACS_SPIN -> ACS_SAFE [order 1] : [energy_low || ~spin_feasible ||...
      |  ~spin_axis_available]
  ACS_SLEW_FAST -> ACS_SAFE [order 2] : [energy_low || ~detumbled ||...
      |  actual_ephem == uint8(0)]
  data: desired_acs input uint8; actual_ephem input uint8; detumbled input boolean; reference_available input boolean; energy_low input boolean; recovery_ready input boolean; wheels_saturated input boolean; desaturated input boolean; spin_feasible input boolean; spin_axis_available input boolean; optical_target_available input boolean; sun_sensor_valid input boolean; actual_acs output uint8 =0

== stateflow chart ADCS_v1/Subsystem2/Mode manager/Mode Manager/ADS_Manager ==
  state ADS_IDLE
    entry:
    actual_ads = uint8(0);
  state ADS_UKF_FINE
    entry:
    actual_ads = uint8(2);
  state ADS_UKF_COARSE
    entry:
    actual_ads = uint8(1);
  ADS_UKF_FINE -> ADS_IDLE [order 2] : [desired_ads == uint8(0) || ads_fault]
  ADS_IDLE -> ADS_UKF_FINE [order 2] : [desired_ads == uint8(2) &&...
      |  ads_fine_allowed && ~ads_fault]
  (default) -> ADS_IDLE
  ADS_UKF_COARSE -> ADS_IDLE [order 1] : [desired_ads == uint8(0) || ads_fault]
  ADS_IDLE -> ADS_UKF_COARSE [order 1] : [desired_ads == uint8(1) ||...
      |  (desired_ads == uint8(2) &&...
      |  ~ads_fine_allowed)]
  ADS_UKF_FINE -> ADS_UKF_COARSE [order 1] : [desired_ads == uint8(1) ||...
      |  ~ads_fine_allowed]
  ADS_UKF_COARSE -> ADS_UKF_FINE [order 2] : [desired_ads == uint8(2) &&...
      |  ads_fine_allowed && ~ads_fault]
  data: desired_ads input uint8; ads_fine_allowed input boolean; ads_fault input boolean; actual_ads output uint8 =0

== stateflow chart ADCS_v1/Subsystem2/Mode manager/Mode Manager/Ephemeris_Manager ==
  state EPHEM_IDLE
    entry:
    actual_ephem = uint8(0);
  state EPHEM_GPS
    entry:
    actual_ephem = uint8(2);
  state EPHEM_TLE
    entry:
    actual_ephem = uint8(1);
  EPHEM_GPS -> EPHEM_IDLE [order 1] : [desired_ephem == uint8(0)]
  EPHEM_IDLE -> EPHEM_GPS [order 2] : [desired_ephem == uint8(2)...
      |  && gps_valid]
  (default) -> EPHEM_IDLE
  EPHEM_IDLE -> EPHEM_TLE [order 1] : [desired_ephem == uint8(1) ||...
      |  (desired_ephem == uint8(2) &&...
      |  ~gps_valid && ~tle_error_high)]
  EPHEM_TLE -> EPHEM_IDLE [order 1] : [desired_ephem == uint8(0)...
      |  || tle_error_high]
  EPHEM_GPS -> EPHEM_TLE [order 2] : [desired_ephem == uint8(1) ||...
      |  ~gps_valid]
  EPHEM_TLE -> EPHEM_GPS [order 2] : [desired_ephem == uint8(2) && gps_valid]
  data: desired_ephem input uint8; gps_valid input boolean; tle_error_high input boolean; actual_ephem output uint8 =0

== stateflow chart ADCS_v1/Subsystem2/Mode manager/Mode Manager/Frame_Manager ==
  state FRAME_INERTIAL
    entry:
    actual_frame = uint8(2);
  state FRAME_LVLH
    entry:
    actual_frame = uint8(3);
  state FRAME_BODY
    entry:
    actual_frame = uint8(1);
  state FRAME_EARTH_TARGET
    entry:
    actual_frame = uint8(4);
  state FRAME_IDLE
    entry:
    actual_frame = uint8(0);
  state FRAME_IMAGING_TDI
    entry:
    actual_frame = uint8(6);
  state FRAME_VNB
    entry:
    actual_frame = uint8(5);
  FRAME_INERTIAL -> (junction 11) : [desired_frame ~= uint8(2)]
  (junction 11) -> FRAME_INERTIAL [order 3] : [desired_frame == uint8(2)]
  FRAME_LVLH -> (junction 11) : [desired_frame ~= uint8(3)]
  (junction 11) -> FRAME_LVLH [order 4] : [desired_frame == uint8(3)]
  FRAME_BODY -> (junction 11) : [desired_frame ~= uint8(1)]
  (junction 11) -> FRAME_BODY [order 2] : [desired_frame == uint8(1)]
  FRAME_EARTH_TARGET -> (junction 11) : [desired_frame ~= uint8(4)]
  (junction 11) -> FRAME_EARTH_TARGET [order 5] : [desired_frame == uint8(4)]
  (junction 11) -> FRAME_IDLE [order 1] : [desired_frame == uint8(0)]
  FRAME_IDLE -> (junction 11) : [desired_frame ~= uint8(0)]
  FRAME_IMAGING_TDI -> (junction 11) : [desired_frame ~= uint8(6)]
  (junction 11) -> FRAME_VNB [order 6] : [desired_frame == uint8(5)]
  (junction 11) -> FRAME_IMAGING_TDI [order 7] : [desired_frame == uint8(6)]
  FRAME_VNB -> (junction 11) : [desired_frame ~= uint8(5)]
  (default) -> FRAME_IDLE
  data: desired_frame input uint8; actual_frame output uint8 =0

== stateflow chart ADCS_v1/Subsystem2/Mode manager/Mode Manager/Mission_Mode_Manager ==
  state M_DETUMBLE
    entry:
    desired_ephem = uint8(0);
    desired_ads = uint8(1);
    desired_frame = uint8(0);
    desired_acs = uint8(1);
    %desired_actuator = uint8(3);
  state M_SAFE_SUN
    entry:
    desired_ephem = uint8(0);
    desired_ads = uint8(0);
    desired_frame = uint8(0);
    desired_acs = uint8(9);
    %desired_actuator = uint8(2);
  state M_Y_SPIN
    entry:
    desired_ephem = uint8(2);
    desired_ads = uint8(1);
    desired_frame = uint8(3);
    desired_acs = uint8(6);
    %desired_actuator = uint8(2);
  state M_IDLE
    entry:
    desired_ephem = uint8(0);
    desired_ads = uint8(0);
    desired_frame = uint8(0);
    desired_acs = uint8(0);
    %desired_actuator = uint8(0);
  state M_MINMAX_DRAG
    entry:
    desired_ephem = uint8(2);
    desired_ads = uint8(2);
    desired_frame = uint8(3);
    %desired_frame = uint8(3 + 2 * drag_use_vnb);
    desired_acs = uint8(2);
    %desired_actuator = uint8(2);
  state M_POINT_NADIR
    entry:
    desired_ephem = uint8(2);
    desired_ads = uint8(2);
    desired_frame = uint8(3);
    desired_acs = uint8(2);
    %desired_actuator = uint8(2);
  state M_SLEW_FIXED
    entry:
    desired_ephem = uint8(2);
    desired_ads = uint8(2);
    desired_frame = uint8(2);
    desired_acs = uint8(4);
    %desired_actuator = uint8(2);
  state M_SLEW_FASTEST
    entry:
    desired_ephem = uint8(2);
    desired_ads = uint8(2);
    desired_frame = uint8(2);
    desired_acs = uint8(5);
    %desired_actuator = uint8(3);
  state M_POINT_MOON
    entry:
    desired_ephem = uint8(2);
    desired_ads = uint8(2);
    desired_frame = uint8(2);
    desired_acs = uint8(2);
    %desired_actuator = uint8(2);
  state M_TDI
    entry:
    desired_ephem = uint8(2);
    desired_ads = uint8(2);
    desired_frame = uint8(6);
    desired_acs = uint8(2);
    %desired_actuator = uint8(2);
  state M_POINT_SUN
    entry:
    desired_ephem = uint8(2);
    desired_ads = uint8(2);
    desired_frame = uint8(2);
    desired_acs = uint8(3);
    %desired_actuator = uint8(2);
  state M_INTERSAT_TRACK
    entry:
    desired_ephem = uint8(2);
    desired_ads = uint8(2);
    desired_frame = uint8(2);
    desired_acs = uint8(2 + 6 * intersat_sensor_tracking);
    %desired_actuator = uint8(2);
  M_DETUMBLE -> (junction 28) : [mission_cmd ~= uint8(1)]
  (junction 28) -> M_DETUMBLE [order 2] : [mission_cmd == uint8(1)]
  M_Y_SPIN -> (junction 28) : [mission_cmd ~= uint8(3)]
  M_SAFE_SUN -> (junction 28) : [mission_cmd ~= uint8(2)]
  (junction 28) -> M_SAFE_SUN [order 3] : [mission_cmd == uint8(2)]
  M_IDLE -> (junction 28) : [mission_cmd ~= uint8(0)]
  (default) -> M_IDLE
  (junction 28) -> M_IDLE [order 1] : [mission_cmd == uint8(0)]
  (junction 28) -> M_Y_SPIN [order 4] : [mission_cmd == uint8(3)]
  (junction 28) -> M_MINMAX_DRAG [order 12] : [mission_cmd == uint8(11)]
  M_MINMAX_DRAG -> (junction 28) : [mission_cmd ~= uint8(11)]
  (junction 28) -> M_POINT_NADIR [order 5] : [mission_cmd == uint8(4)]
  M_POINT_NADIR -> (junction 28) : [mission_cmd ~= uint8(4)]
  (junction 28) -> M_SLEW_FIXED [order 8] : [mission_cmd == uint8(7)]
  M_SLEW_FASTEST -> (junction 28) : [mission_cmd ~= uint8(8)]
  (junction 28) -> M_SLEW_FASTEST [order 9] : [mission_cmd == uint8(8)]
  M_SLEW_FIXED -> (junction 28) : [mission_cmd ~= uint8(7)]
  (junction 28) -> M_POINT_MOON [order 7] : [mission_cmd == uint8(6)]
  (junction 28) -> M_POINT_SUN [order 6] : [mission_cmd == uint8(5)]
  M_POINT_MOON -> (junction 28) : [mission_cmd ~= uint8(6)]
  M_POINT_SUN -> (junction 28) : [mission_cmd ~= uint8(5)]
  (junction 28) -> M_INTERSAT_TRACK [order 10] : [mission_cmd == uint8(9)]
  (junction 28) -> M_TDI [order 11] : [mission_cmd == uint8(10)]
  M_INTERSAT_TRACK -> (junction 28) : [mission_cmd ~= uint8(9)]
  M_TDI -> (junction 28) : [mission_cmd ~= uint8(10)]
  data: mission_cmd input uint8; intersat_sensor_tracking input boolean; desired_ephem output uint8 =0; desired_ads output uint8 =0; desired_frame output uint8 =0; desired_acs output uint8 =0

== stateflow chart ADCS_v1/Subsystem2/Mode manager/Status_Manager ==
  state STATUS
    during:
    mode_degraded = (actual_ephem ~= desired_ephem) || (actual_ads ~= desired_ads) || (actual_frame ~= desired_frame) || (actual_acs ~= desired_acs);
  (default) -> STATUS
  data: desired_ephem input uint8; desired_ads input uint8; desired_frame input uint8; desired_acs input uint8; actual_ephem input uint8; actual_ads input uint8; actual_frame input uint8; actual_acs input uint8; mode_degraded output boolean =0

== matlab function ADCS_v1/Subsystem1/Controller/Control Algorithms/RW Torque Commands/OPTICAL/MATLAB Function2 ==
  data: y_cm output; x_cm output; u input
function [y_cm,x_cm] = fcn(u)
% u(u>5) = uint8(255);
% y = zeros(size(u,1),size(u,2));
% for i = 1:size(u,1)
%     for j = 1:size(u,2)
%         y(i,j) = double(max(u(i,j,:)));
%     end
% end
% S = sum(sum(y));
% if S == 0
%     x_cm = 0;
%     y_cm = 0;
% else
%     x_cm = sum(sum(y.*(1:size(y,2)),2))/S - size(y,2)/2;
%     y_cm = sum(sum(y.*(1:size(y,1))',1))/S- size(y,1)/2;
% end

y = double(max(u, [], 3));

% Binary foreground
bw = y > 5;

% Connected components
CC = bwconncomp(bw, 8);

if CC.NumObjects == 0
    x_cm = 0;
    y_cm = 0;
else
    % Calculate area of every component
    areas = cellfun(@numel, CC.PixelIdxList);

    % Largest connected component = satellite
    [~, idx] = max(areas);

    satelliteMask = false(size(bw));
    satelliteMask(CC.PixelIdxList{idx}) = true;

    % Geometric centroid
    [r, c] = find(satelliteMask);

    x_cm = mean(c) - size(y,2)/2;
    y_cm = mean(r) - size(y,1)/2;
end

== stateflow chart ADCS_v1/Subsystem1/Mode manager/Mode Manager/ACS_Manager ==
  state ACS_DETUMBLE
    entry:
    actual_acs = uint8(1);
    exit:
    if desired_acs == uint8(1)
    desired_acs == uint8(0)
    end
  state ACS_POINT
    entry:
    actual_acs = uint8(2);
  state ACS_IDLE
    entry:
    actual_acs = uint8(0);
  state ACS_DESAT
    entry:
    actual_acs = uint8(4);
    exit:
    if desired_acs == uint8(4)
    desired_acs == uint8(0)
    end
  state ACS_OPTICAL
    entry:
    actual_acs = uint8(5);
  state ACS_SPIN
    entry:
    actual_acs = uint8(3);
  state ACS_SAFE
    entry:
    actual_acs = uint8(6);
  ACS_OPTICAL -> ACS_POINT [order 3] : [~optical_target_available &&...
      |  ~energy_low]
  (junction 25) -> ACS_DETUMBLE [order 2] : [(desired_acs == uint8(1)&&desaturated)  ...
      | ||~detumbled]
  ACS_DETUMBLE -> (junction 25) : [ zero_omega]
  ACS_POINT -> ACS_SAFE [order 2] : [energy_low || ~reference_available ||...
      |  actual_ephem == uint8(0)]%~detumbled ||
  ACS_POINT -> (junction 25) [order 1] : [desired_acs ~= uint8(2) ||...
      | ~detumbled]
  (junction 25) -> ACS_POINT [order 3] : [desired_acs == uint8(2) && detumbled && desaturated]
  (default) -> ACS_IDLE
  (junction 25) -> ACS_IDLE [order 1] : [desired_acs == uint8(0) && detumbled && desaturated]
  ACS_IDLE -> (junction 25) : [desired_acs ~= uint8(0)]
  ACS_DESAT -> (junction 25) [order 1] : [desaturated ]%&& recovery_ready &&~energy_low
  (junction 25) -> ACS_DESAT [order 5] : [desired_acs == uint8(4)||wheels_saturated]
  (junction 25) -> ACS_OPTICAL [order 6] : [desired_acs == uint8(5)]
  ACS_OPTICAL -> (junction 25) [order 1] : [desired_acs ~= uint8(5) && optical_target_available]
  ACS_SAFE -> (junction 25) : [desired_acs ~= uint8(9) &&...
      |  ~energy_low && recovery_ready &&...
      |  sun_sensor_valid && ~((desired_acs == uint8(2)) &&...
      |  ~reference_available) && ~((desired_acs == uint8(6)) &&...
      |  (~spin_feasible || ~spin_axis_available))]
  (junction 25) -> ACS_SAFE [order 7] : [desired_acs == uint8(9)]
  (junction 25) -> ACS_SPIN [order 4] : [desired_acs == uint8(3)]
  ACS_SPIN -> (junction 25) [order 2] : [desired_acs ~= uint8(3)]
  ACS_DESAT -> ACS_SAFE [order 2] : [energy_low]
  ACS_OPTICAL -> ACS_SAFE [order 2] : [energy_low]
  ACS_SPIN -> ACS_SAFE [order 1] : [energy_low || ~spin_feasible ||...
      |  ~spin_axis_available]
  data: desired_acs input uint8; actual_ephem input uint8; detumbled input boolean; zero_omega input; reference_available input boolean; energy_low input boolean; recovery_ready input boolean; wheels_saturated input boolean; desaturated input boolean; spin_feasible input boolean; spin_axis_available input boolean; optical_target_available input boolean; sun_sensor_valid input boolean; actual_acs output uint8 =0
